simulink model "ecu_crank"  (R2026a)
settings: Solver=FixedStepDiscrete  StopTime=10  FixedStep=0.001  SampleTimeConstraint=STIndependent
Description:
  | Crank decoder and cam-wheel learning. Source of truth for firmware/gen/ecu_crank.
settings Model: Creator=jj1001000  LastModifiedBy=jj1001000
settings OptimizationCC: DefaultUnderspecifiedDataType=single
settings DebuggingCC: ParameterPrecisionLossMsg=none
settings HardwareCC: ProdLargestAtomicInteger=Long  ProdLargestAtomicFloat=Double  ProdHWDeviceType=ARM Compatible->ARM Cortex-M
settings RTWCC: SystemTargetFile=ert.tlc  GenCodeOnly=on  Description=Embedded Coder
settings ERTTargetCC: UtilityFuncGeneration=Shared location  IncludeMdlTerminateFcn=off  CodeInterfacePackaging=Reusable function  SupportNonFinite=off

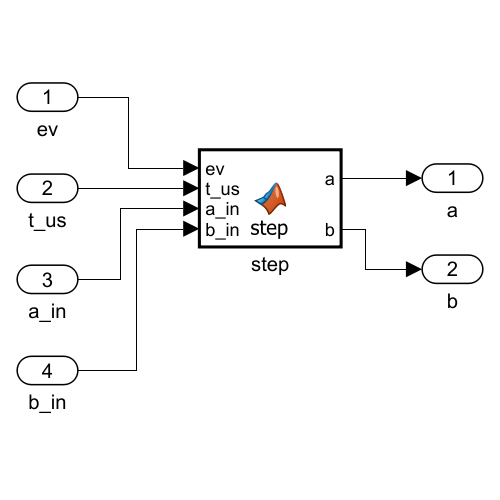
[thumbnail: Simulink's stored preview of the top-level diagram]
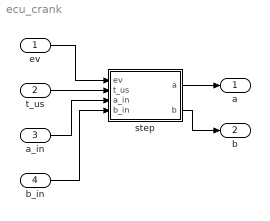
== system ecu_crank ==
  ev : Inport  OutDataTypeStr=uint8
  t_us : Inport  Port=2  OutDataTypeStr=uint32
  a_in : Inport  Port=3  OutDataTypeStr=uint32  PortDimensions=8
  b_in : Inport  Port=4  OutDataTypeStr=uint8  PortDimensions=33
  step : MATLAB Function  TreatAsAtomicUnit=on
  a : Outport  OutDataTypeStr=uint32
  b : Outport  Port=2  OutDataTypeStr=uint8
  wires:
  ev/1 -> step/1(ev)
  b_in/1 -> step/4(b_in)
  a_in/1 -> step/3(a_in)
  t_us/1 -> step/2(t_us)
  step/1(a) -> a/1
  step/2(b) -> b/1

== matlab function ecu_crank/step ==
  data: ev input uint8; a output uint32; t_us input uint32; a_in input uint32; b_in input uint8; b output uint8
function [a, b] = step(ev, t_us, a_in, b_in)
%#codegen
a = a_in; b = b_in;
EDGES = uint8(58); WIN = uint8(6); TMO = uint32(50000); TOL = uint8(2); MISS = uint8(2);
F_GAP = uint8(1); F_TMO = uint8(2);
if ev == uint8(0)
    if b(9) == 0                                    % have
        b(9) = uint8(1); a(1) = t_us;
    else
        period = since(t_us, a(1));
        if period > TMO
            b = lose(b, F_TMO);
            a(2) = uint32(0); b(7) = uint8(0); b(8) = uint8(0);   % prev_period, nper, head
            b(11) = uint8(0); b(10) = uint8(0); b(16) = uint8(0); % gap_seen, count, prev_gap
            a(1) = t_us;
        else
            if b(16) ~= 0
                tp = idivide(a(2), uint32(3), 'floor');
            else
                tp = a(2);
            end
            if ~(period < idivide(tp, uint32(2), 'floor'))    % else noise: dropped, no change
                gap = a(2) ~= 0 && period > a(2) + idivide(a(2), uint32(2), 'floor');
                hd = int32(b(8));
                a(3 + hd) = period;
                if gap
                    b(1 + hd) = uint8(18);
                else
                    b(1 + hd) = uint8(6);
                end
                b(8) = uint8(mod(hd + int32(1), int32(WIN)));
                if b(7) < WIN, b(7) = b(7) + uint8(1); end
                if gap
                    in_place = b(11) ~= 0 && b(10) == EDGES - uint8(1);
                    if ~in_place
                        b = lose(b, F_GAP);
                    elseif b(12) == 0
                        b(12) = uint8(1);
                    end
                    b(11) = uint8(1); b(10) = uint8(0);
                    b = cam_at_gap(b, in_place, TOL, MISS);
                    b(17) = uint8(0); b(18) = uint8(0); b(19) = uint8(0);
                else
                    b(10) = uint8(mod(int32(b(10)) + int32(1), int32(256)));   % uint8 wraps, as in C
                    if b(10) >= EDGES
                        b = lose(b, F_GAP);
                        b(11) = uint8(0);
                    end
                end
                a(1) = t_us; a(2) = period; b(16) = uint8(gap);
            end
        end
    end
elseif ev == uint8(1)
    if b(17) == 0, b(18) = b(10); end
    b(19) = b(10);
    if b(17) < uint8(255), b(17) = b(17) + uint8(1); end
elseif ev == uint8(2)
    d = since(t_us, a(1));
    % as C's (int32_t)(t - last) > TIMEOUT: over it, and positive as a signed value
    if b(12) ~= 0 && d > TMO && d <= uint32(2147483647)
        b = lose(b, F_TMO);
    end
end

function d = since(t, last)                      % t - last, wrapping as uint32_t does
if t >= last
    d = t - last;
else
    d = (t + (intmax('uint32') - last)) + uint32(1);   % neither sum can saturate
end

function b = lose(b, why)
if b(12) ~= 0, b(15) = why; end
b(12) = uint8(0); b(13) = uint8(0); b(7) = uint8(0);

function y = near(x, z, TOL)
if x > z
    y = (x - z) <= TOL;
else
    y = (z - x) <= TOL;
end

function y = sig_match(s, r, TOL)                % s, r: [n first last]
y = s(1) == r(1) && (s(1) == 0 || (near(s(2), r(2), TOL) && near(s(3), r(3), TOL)));

function k = sig_marker(s, r, TOL)               % 1: s, 0: r, -1: too alike
if s(1) ~= r(1)
    k = int8(s(1) > r(1));
elseif s(1) == 0
    k = int8(-1);
elseif ~near(s(2), r(2), TOL)
    k = int8(s(2) < r(2));
elseif ~near(s(3), r(3), TOL)
    k = int8(s(3) < r(3));
else
    k = int8(-1);
end

function b = cam_at_gap(b, whole, TOL, MISS)
% b(17:19) cur, 20:22 prev, 23:25 mark, 26:28 other; 29 prev_ok, 30 learned,
% 31 proven, 32 miss, 33 clean; 12 synced, 13 phased, 14 rev
if ~whole
    b(29) = uint8(0); b(14) = bitxor(b(14), uint8(1));
    return;
end
nxt = int8(-1); missed = false;
cur = b(17:19); prv = b(20:22);
if b(30) ~= 0
    if sig_match(cur, b(23:25), TOL)
        nxt = int8(0);
    elseif sig_match(cur, b(26:28), TOL)
        nxt = int8(1);
    end
    if nxt < 0
        missed = true; b(33) = uint8(0);
        if b(31) == 0
            b(30) = uint8(0);
        else
            b(32) = uint8(mod(int32(b(32)) + int32(1), int32(256)));
            if b(32) >= MISS, b(30) = uint8(0); end
        end
    else
        b(33) = uint8(mod(int32(b(33)) + int32(1), int32(256)));
        if b(33) >= uint8(2)
            b(33) = uint8(2); b(31) = uint8(1); b(32) = uint8(0);
        end
    end
end
if b(30) == 0 && b(29) ~= 0 && ~missed
    k = sig_marker(cur, prv, TOL);
    if k >= 0
        if k ~= 0
            b(23:25) = cur; b(26:28) = prv; nxt = int8(0);
        else
            b(23:25) = prv; b(26:28) = cur; nxt = int8(1);
        end
        b(30) = uint8(1); b(31) = uint8(0); b(32) = uint8(0); b(33) = uint8(0);
    end
end
if nxt < 0
    b(13) = uint8(0); b(14) = bitxor(b(14), uint8(1));
else
    agrees = b(13) == 0 || b(14) == bitxor(uint8(nxt), uint8(1));
    b(14) = uint8(nxt);
    b(13) = uint8(b(12) ~= 0 && agrees);
end
b(20:22) = cur;
b(29) = uint8(~missed);
